simulink model "model_LMPC_yawVarFakeRelative"  (R2024b)
settings: Solver=VariableStepAuto  StartTime=0.0  StopTime=100  RelTol=1e-3
undefined symbols (not defined in the file): boat, boat_wave_Torque, boatModels, drone, environment, settings
libraries: mpclib x4, sharedtransform x3, utils x1, uavutilslib x1
settings Model: Creator=domac  LastModifiedBy=domac

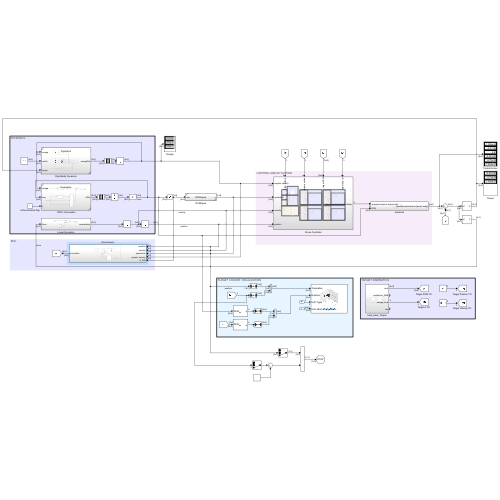
[thumbnail: Simulink's stored preview of the top-level diagram]
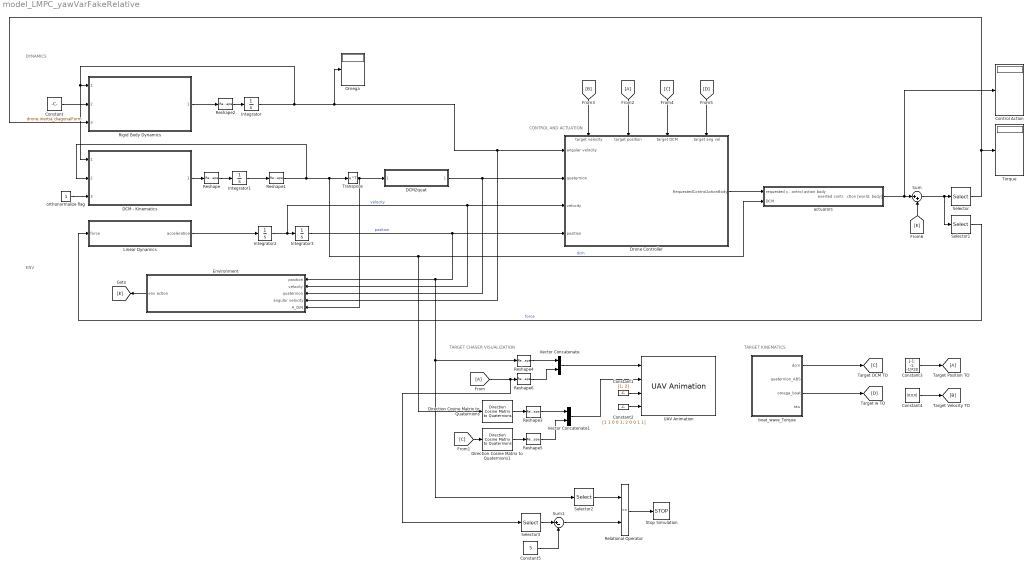
== system model_LMPC_yawVarFakeRelative ==
  note: TARGET CHASER VISUALIZATION
  note: CONTROL AND ACTUATION
  note: DYNAMICS
  note: TARGET KINEMATICS
  note: ENV
  " DCM - Kinematics" : Subsystem  ReferencedSubsystem=Kinematics
  Constant : Constant  Value=drone.inertia_diagonalForm  VectorParams1D=off
  Constant1 : Constant  Value=[1; 2]
  Constant2 : Constant  Value=[1 1 0 0 1; 2 0 0 1 1]
  Constant3 : Constant  Value=[-1; -1; -1]*20
  Constant4 : Constant  Value=[0;0;0]
  Constant5 : Constant  Value=5
  Control Action : Display
  DCM2quat : Subsystem  ReferencedSubsystem=DCM2quat
  Direction Cosine Matrix to Quaternions : sharedtransform/Direction Cosine Matrix  to Quaternions  aMode=0  action=None  tolerance=eps(2)
      settings: LibrarySourceBlock=|
      | aerolibtransform2/Direction Cosine Matrix
      | to Quaternions
  Direction Cosine Matrix to Quaternions1 : sharedtransform/Direction Cosine Matrix  to Quaternions  aMode=0  action=None  tolerance=eps(2)
      settings: LibrarySourceBlock=|
      | aerolibtransform2/Direction Cosine Matrix
      | to Quaternions
  Drone Controller : Subsystem
      settings: PortSchema="{\"entries\":[{\"content\":{\"sides\":[{\"content\":{\"connectorIds\":[\"In1\",\"In2\",\"In3\",\"In4\"]},\"type\":\"ConnectorPlacement.EquallySpacedRectSide\",\"uuid\":\"5cbf5d97-798f-4abe-9063-7d9475aab2f7\"},{\"content\":{\"connectorIds\":[\"Out1\"],\"side\":\"RIGHT\"},\"type\":\"ConnectorPlacement.EquallySpacedRectSide\",\"uuid\":\"8e1c1ff5-210e-451e-9bb4-b2ea9c687a0c\"},{\"content\":{\"connectorIds\":[\"In5\",\"In6\",\"In7\",\"In8\"],\"side\":\"TOP\"},\"type\":\"ConnectorPlacement.EquallySpacedRectSide\",\"uuid\":\"7263c23d-5bc0-464e-848c-51e45572c4cc\"}]},\"type\":\"ConnectorPlacement.EquallySpacedConnector\",\"uuid\":\"7a6c5e6f-7804-4a94-a46d-c2acf2bd8613\"}],\"packageUris\":[\"http://schema.mathworks.com/mf0/Connector/R2020b\"],\"version\":\"1.0\"}"
  Environment : Subsystem
  From : From
  From2 : From
  Integrator : Integrator  InitialCondition=drone.w0
  Integrator1 : Integrator  InitialCondition=[drone.initialDCM(:,1); drone.initialDCM(:,2); drone.initialDCM(:,3)]
  Integrator2 : Integrator  InitialCondition=drone.v0
  Integrator3 : Integrator  InitialCondition=drone.x0
  Linear Dynamics : Subsystem
  Omega : Display
  Relational Operator : RelationalOperator  Operator=<=  OutDataTypeStr=boolean  RndMeth=Simplest  InputSameDT=off
  Reshape : Reshape  OutputDimensionality=Column vector (2-D)
  Reshape1 : Reshape  OutputDimensionality=Customize  OutputDimensions=[3, 3]
  Reshape2 : Reshape  OutputDimensionality=Column vector (2-D)
  Reshape{3..6} (4 alike) : Reshape  OutputDimensionality=Row vector (2-D)
  Rigid Body Dynamics : Subsystem  ReferencedSubsystem=Dynamics
  Selector : Selector  InputPortWidth=6  IndexOptions=Index vector (dialog)  Indices=[4 5 6]  OutputSizes=1
  Selector1 : Selector  InputPortWidth=6  IndexOptions=Index vector (dialog)  Indices=[1 2 3]  OutputSizes=1
  Selector2 : Selector  InputPortWidth=3  IndexOptions=Index vector (dialog)  Indices=3  OutputSizes=1
  Selector3 : Selector  InputPortWidth=3  IndexOptions=Index vector (dialog)  Indices=3  OutputSizes=1
  Stop Simulation : Stop
  Sum : Sum  Inputs=|++
  Sum1 : Sum  Inputs=|+-
  Target Position TO : Goto
  Torque : Display
  Transpose : Math  Operator=transpose
  UAV Animation : uavutilslib/UAV Animation  NumUAV=2  DynamicUAVConfig=on  UAVType=Multirotor  UAVSize=1  UAVColor=[1 0 0]  UAVTrajectoryAlpha=1  InertialZDirection=Up  RotationFormat=Quaternion  DrawMarkers=off  SampleTime=0.2
  Vector Concatenate : Concatenate  Mode=Multidimensional array
  Vector Concatenate1 : Concatenate  Mode=Multidimensional array
  actuarors : Subsystem
  boat_wave_Torque : Subsystem  AncestorBlock=boatModels/boat_wave_Torque
  orthonormalize flag : Constant
  wires:
  Constant/1 -> Rigid Body Dynamics/2
  Integrator1/1 -> Reshape1/1
  DCM2quat/1 -> Drone Controller/2(quaternion), Environment/3(quaternion)
  [D] -> Drone Controller/8(target ang vel)
  Vector Concatenate/1 -> UAV Animation/1
  Reshape4/1 -> Vector Concatenate/1
  From2/1 -> Drone Controller/6(target position)
  Vector Concatenate1/1 -> UAV Animation/2
  orthonormalize flag/1 -> " DCM - Kinematics"/3
  Direction Cosine Matrix to Quaternions/1 -> Reshape3/1
  Sum/1 -> Selector/1, Selector1/1
  Reshape5/1 -> Vector Concatenate1/2
  Reshape6/1 -> Vector Concatenate/2
  actuarors/1(exerted control action [world; body]) -> Control Action/1, Sum/1
  [B] -> Drone Controller/5(target velocity)
  Selector1/1 -> Linear Dynamics/1(force)  "force"
  Reshape/1 -> Integrator1/1
  Reshape1/1 -> " DCM - Kinematics"/2, Direction Cosine Matrix to Quaternions/1, actuarors/2(DCM), Transpose/1  "dcm"
  Constant1/1 -> UAV Animation/3
  [C] -> Drone Controller/7(target DCM)
  [C] -> Direction Cosine Matrix to Quaternions1/1
  Selector/1 -> Rigid Body Dynamics/3, Torque/1
  From/1 -> Selector3/1, Reshape6/1
  Reshape2/1 -> Integrator/1
  Transpose/1 -> Environment/5(A_D/N), DCM2quat/1
  Rigid Body Dynamics/1 -> Reshape2/1
  Integrator3/1 -> Environment/1(position), Reshape4/1, Selector2/1, Drone Controller/4("position ")  "position"
  Integrator2/1 -> Drone Controller/3(velocity), Environment/2(velocity), Integrator3/1  "velocity"
  [E] -> Sum/2
  " DCM - Kinematics"/1 -> Reshape/1
  Environment/1(env action) -> [E]
  Direction Cosine Matrix to Quaternions1/1 -> Reshape5/1
  Integrator/1 -> " DCM - Kinematics"/1, Rigid Body Dynamics/1, Omega/1, Drone Controller/1(angular velocity), Environment/4(angular velocity)
  Reshape3/1 -> Vector Concatenate1/1
  Linear Dynamics/1(acceleration) -> Integrator2/1
  Constant2/1 -> UAV Animation/4
  boat_wave_Torque/1(dcm) -> [C]
  boat_wave_Torque/3(omega_boat) -> [D]
  Constant4/1 -> [B]
  Constant3/1 -> Target Position TO/1
  Drone Controller/1(RequestedControlActionBody) -> actuarors/1(requested control action body)
  Selector2/1 -> Relational Operator/1
  Selector3/1 -> Sum1/1
  Constant5/1 -> Sum1/2
  Sum1/1 -> Relational Operator/2
  Relational Operator/1 -> Stop Simulation/1

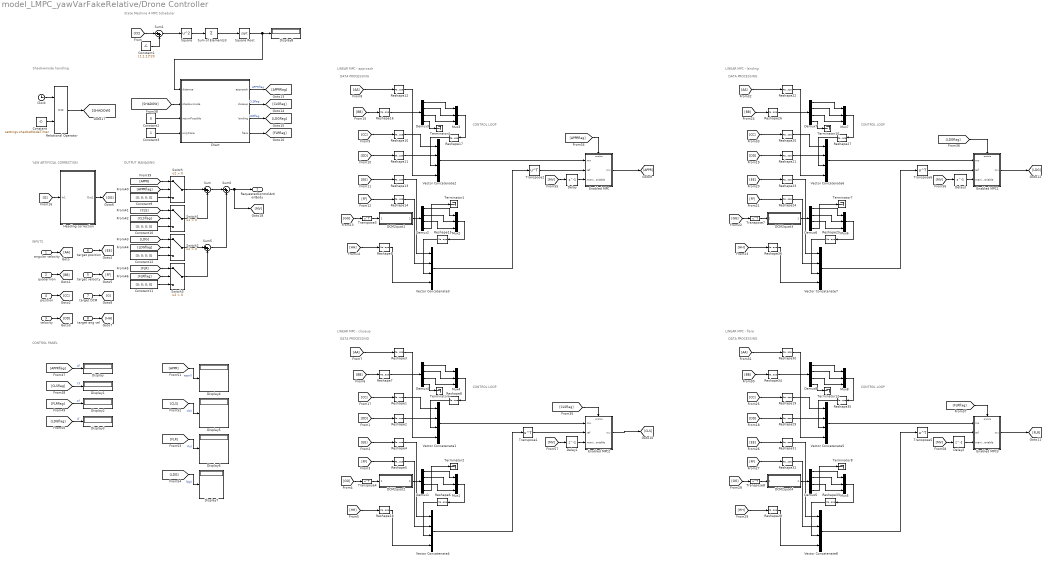
== system model_LMPC_yawVarFakeRelative/Drone Controller ==
  note: CONTROL PANEL
  note: OUTPUT MANAGING
  note: Shadowmode handling
  note: State Machine 4 MPC Scheduler
  note: YAW ARTIFICIAL CORRECTION
  note: INPUTS
  note: DATA PROCESSING
  note: CONTROL LOOP
  note: LINEAR MPC - approach
  note: DATA PROCESSING
  note: CONTROL LOOP
  note: LINEAR MPC - closeup
  note: LINEAR MPC - flare
  note: DATA PROCESSING
  note: CONTROL LOOP
  note: DATA PROCESSING
  note: CONTROL LOOP
  note: LINEAR MPC - landing
  angular velocity : Inport
  quaternion : Inport  Port=2
  velocity : Inport  Port=3
  "position " : Inport  Port=4
  target velocity : Inport  Port=5
  target position : Inport  Port=6
  target DCM : Inport  Port=7
  target ang vel : Inport  Port=8
  Chart : Stateflow chart  TreatAsAtomicUnit=on
  Clock : Clock
  Constant : Constant  Value=settings.shadowModeTimer
  Constant1 : Constant  Value=[1;1;1]*20
  Constant{9..12} (4 alike) : Constant  Value=[0; 0; 0; 0]
  Constant2 : Constant  Value=0
  Constant3 : Constant
  DCM2quat{1..4} (4 alike) : Subsystem  ReferencedSubsystem=DCM2quat
  Delay{,1..3} (4 alike) : Delay  DelayLength=1
  Demux{1..8} (8 alike) : Demux
  Display{,1..8} (9 alike) : Display
  Enabled MPC : Subsystem  TreatAsAtomicUnit=on
  Enabled MPC1 : Subsystem  TreatAsAtomicUnit=on
  Enabled MPC2 : Subsystem  TreatAsAtomicUnit=on
  Enabled MPC3 : Subsystem  TreatAsAtomicUnit=on
  Heading correction : Subsystem
  Mux{1..8} (8 alike) : Mux  Inputs=3
  Relational Operator : RelationalOperator  Operator=<=  OutDataTypeStr=boolean  RndMeth=Simplest  InputSameDT=off
  Reshape{1..36} (36 alike) : Reshape  OutputDimensionality=Column vector (2-D)
  Square : Math  Operator=square
  Square Root : Sqrt
  Sum{,1,5..6} (4 alike) : Sum  Inputs=|++
  Sum of Elements3 : Sum  Inputs=+
  Switch{,1..3} (4 alike) : Switch  Criteria=u2 > Threshold  SaturateOnIntegerOverflow=off  InputSameDT=off
  Terminator{1..2,4,6..8,10,12} (8 alike) : Terminator
  Transpose{1..8} (8 alike) : Math  Operator=transpose
  Vector Concatenate{1..8} (8 alike) : Concatenate  NumInputs=4
  RequestedControlActionBody : Outport
  wires:
  Transpose2/1 -> Enabled MPC/2(ref)
  Vector Concatenate2/1 -> Enabled MPC/1(mo)
  [FF] -> Reshape14/1
  Demux2/2 -> Mux2/2
  Reshape10/1 -> Vector Concatenate2/1
  Reshape12/1 -> Vector Concatenate2/4
  Reshape15/1 -> Vector Concatenate3/3
  [HH] -> Reshape9/1
  Vector Concatenate3/1 -> Transpose2/1
  Reshape9/1 -> Vector Concatenate3/4
  Demux2/1 -> Mux2/1
  [CC] -> Reshape10/1
  DCM2quat1/1 -> Demux2/1
  [BB] -> Reshape16/1
  Reshape11/1 -> Vector Concatenate2/2
  Reshape17/1 -> Vector Concatenate2/3
  [DD] -> Reshape11/1
  Reshape14/1 -> Vector Concatenate3/2
  Mux3/1 -> Reshape17/1
  [EE] -> Reshape13/1
  Mux2/1 -> Reshape15/1
  Reshape16/1 -> Demux3/1
  Demux3/1 -> Mux3/1
  [AA] -> Reshape12/1
  Demux3/4 -> Terminator4/1
  Demux3/3 -> Mux3/3
  Demux2/4 -> Terminator1/1
  Transpose3/1 -> DCM2quat1/1
  Demux3/2 -> Mux3/2
  Reshape13/1 -> Vector Concatenate3/1
  Demux2/3 -> Mux2/3
  angular velocity/1 -> [AA]
  quaternion/1 -> [BB]
  velocity/1 -> [DD]
  "position "/1 -> [CC]
  target position/1 -> [EE]
  target velocity/1 -> [FF]
  target ang vel/1 -> [HH]
  [GG] -> Transpose3/1
  target DCM/1 -> [G]
  [G] -> Heading correction/1(In1)
  Heading correction/1(Out1) -> [GG]
  Enabled MPC/1(mv) -> [APPR]
  Vector Concatenate1/1 -> Enabled MPC2/1(mo)
  DCM2quat2/1 -> Demux1/1
  [BB] -> Reshape7/1
  Transpose1/1 -> Enabled MPC2/2(ref)
  Reshape8/1 -> Vector Concatenate1/3
  Enabled MPC2/1(mv) -> [CLS]
  [GG] -> Transpose4/1
  [CC] -> Reshape1/1
  Demux4/4 -> Terminator6/1
  [HH] -> Reshape18/1
  Demux1/4 -> Terminator2/1
  Reshape6/1 -> Vector Concatenate4/3
  Demux4/3 -> Mux4/3
  Demux4/2 -> Mux4/2
  Mux4/1 -> Reshape8/1
  [EE] -> Reshape4/1
  Reshape7/1 -> Demux4/1
  Demux1/2 -> Mux1/2
  Transpose4/1 -> DCM2quat2/1
  Mux1/1 -> Reshape6/1
  [FF] -> Reshape5/1
  Reshape5/1 -> Vector Concatenate4/2
  Reshape3/1 -> Vector Concatenate1/4
  Reshape1/1 -> Vector Concatenate1/1
  Reshape2/1 -> Vector Concatenate1/2
  Demux1/3 -> Mux1/3
  [DD] -> Reshape2/1
  Reshape4/1 -> Vector Concatenate4/1
  Vector Concatenate4/1 -> Transpose1/1
  Demux4/1 -> Mux4/1
  Reshape18/1 -> Vector Concatenate4/4
  [AA] -> Reshape3/1
  Demux1/1 -> Mux1/1
  Vector Concatenate6/1 -> Enabled MPC1/1(mo)
  Enabled MPC1/1(mv) -> [LDG]
  Demux5/1 -> Mux5/1
  [AA] -> Reshape30/1
  Transpose6/1 -> Enabled MPC1/2(ref)
  Demux5/3 -> Mux5/3
  [DD] -> Reshape29/1
  Demux8/1 -> Mux8/1
  Reshape31/1 -> Vector Concatenate8/1
  Vector Concatenate8/1 -> Transpose5/1
  Reshape30/1 -> Vector Concatenate5/4
  Mux5/1 -> Reshape33/1
  Demux8/3 -> Mux8/3
  Demux5/2 -> Mux5/2
  Reshape28/1 -> Vector Concatenate8/4
  Mux8/1 -> Reshape35/1
  [FF] -> Reshape32/1
  [CC] -> Reshape19/1
  Reshape19/1 -> Vector Concatenate5/1
  [BB] -> Reshape34/1
  DCM2quat4/1 -> Demux5/1
  DCM2quat3/1 -> Demux6/1
  Reshape33/1 -> Vector Concatenate8/3
  Reshape35/1 -> Vector Concatenate5/3
  [BB] -> Reshape26/1
  Reshape27/1 -> Vector Concatenate6/3
  [GG] -> Transpose7/1
  Demux8/2 -> Mux8/2
  [CC] -> Reshape20/1
  Demux7/4 -> Terminator10/1
  Transpose8/1 -> DCM2quat4/1
  [HH] -> Reshape28/1
  [HH] -> Reshape36/1
  Demux8/4 -> Terminator12/1
  Reshape29/1 -> Vector Concatenate5/2
  Demux6/4 -> Terminator7/1
  Reshape25/1 -> Vector Concatenate7/3
  Demux7/3 -> Mux7/3
  [EE] -> Reshape31/1
  Demux7/2 -> Mux7/2
  Mux7/1 -> Reshape27/1
  [EE] -> Reshape23/1
  Vector Concatenate5/1 -> Enabled MPC3/1(mo)
  Reshape26/1 -> Demux7/1
  Reshape34/1 -> Demux8/1
  Transpose5/1 -> Enabled MPC3/2(ref)
  Demux6/2 -> Mux6/2
  Transpose7/1 -> DCM2quat3/1
  Mux6/1 -> Reshape25/1
  [FF] -> Reshape24/1
  Reshape24/1 -> Vector Concatenate7/2
  Reshape22/1 -> Vector Concatenate6/4
  Reshape20/1 -> Vector Concatenate6/1
  Reshape21/1 -> Vector Concatenate6/2
  Enabled MPC3/1(mv) -> [FLR]
  Demux6/3 -> Mux6/3
  [DD] -> Reshape21/1
  Reshape23/1 -> Vector Concatenate7/1
  Vector Concatenate7/1 -> Transpose6/1
  [GG] -> Transpose8/1
  Demux7/1 -> Mux7/1
  Demux5/4 -> Terminator8/1
  Reshape36/1 -> Vector Concatenate7/4
  [AA] -> Reshape22/1
  Reshape32/1 -> Vector Concatenate8/2
  Demux6/1 -> Mux6/1
  Chart/1(approach) -> [APPRflag]  "APPRflag"
  Chart/2(closeup) -> [CLSflag]  "CLSflag"
  Chart/3(landing) -> [LDGflag]  "LDGflag"
  Chart/4(flare) -> [FLRflag]
  [APPRflag] -> Enabled MPC/Enable
  [CLSflag] -> Enabled MPC2/Enable
  [LDGflag] -> Enabled MPC1/Enable
  [FLRflag] -> Enabled MPC3/Enable
  [SHADOW] -> Chart/2(shadowmode)
  Clock/1 -> Relational Operator/1
  Constant/1 -> Relational Operator/2
  Relational Operator/1 -> [SHADOW]
  [APPR] -> Switch/1
  [APPRflag] -> Switch/2
  Constant9/1 -> Switch/3
  [CLS] -> Switch1/1
  [CLSflag] -> Switch1/2
  Constant10/1 -> Switch1/3
  [LDG] -> Switch2/1
  Constant11/1 -> Switch3/3
  [FLR] -> Switch3/1
  [LDGflag] -> Switch2/2
  [FLRflag] -> Switch3/2
  Constant12/1 -> Switch2/3
  Switch/1 -> Sum/1
  Switch1/1 -> Sum/2
  Switch3/1 -> Sum5/2
  Switch2/1 -> Sum5/1
  Sum/1 -> Sum6/1
  Sum5/1 -> Sum6/2
  Sum6/1 -> [MV], RequestedControlActionBody/1
  Square/1 -> Sum of Elements3/1
  Sum of Elements3/1 -> Square Root/1
  Square Root/1 -> Display8/1, Chart/1(distance)
  [APPRflag] -> Display/1  "Af"
  [CLSflag] -> Display1/1  "Cf"
  [FLRflag] -> Display2/1  "Ff"
  [LDGflag] -> Display3/1  "Lf"
  [LDG] -> Display7/1  "ldgU"
  [FLR] -> Display6/1  "flrU"
  [APPR] -> Display4/1  "apprU"
  [CLS] -> Display5/1  "clsU"
  [CC] -> Sum1/1
  Sum1/1 -> Square/1
  Constant1/1 -> Sum1/2
  [MV] -> Delay/1
  [MV] -> Delay3/1
  [MV] -> Delay1/1
  [MV] -> Delay2/1
  Delay/1 -> Enabled MPC/3(manipulated variable)
  Delay1/1 -> Enabled MPC2/3(manipulated variable)
  Delay2/1 -> Enabled MPC3/3(manipulated variable)
  Delay3/1 -> Enabled MPC1/3(manipulated variable)
  Constant2/1 -> Chart/3(returnPossible)
  Constant3/1 -> Chart/4(onlyFlare)

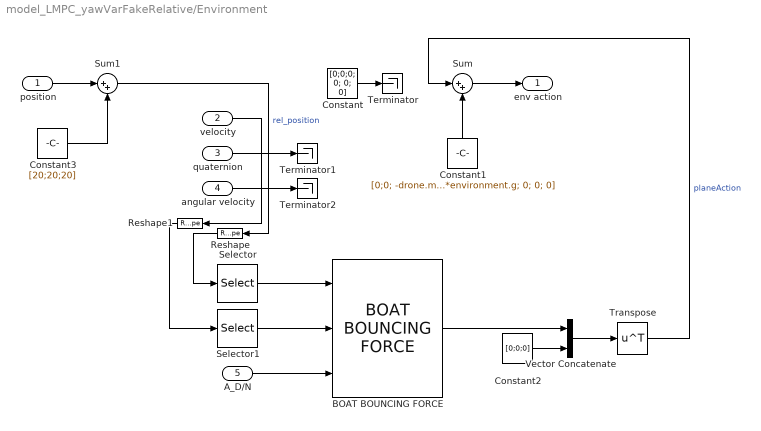
== system model_LMPC_yawVarFakeRelative/Environment ==
  position : Inport
  velocity : Inport  Port=2
  quaternion : Inport  Port=3
  angular velocity : Inport  Port=4
  A_D/N : Inport  Port=5
  BOAT BOUNCING FORCE : utils/BOAT BOUNCING FORCE  SystemSampleTime=-1  VariantActivationTime=update diagram  AllowFlexibleInterface=on  Latency=0  AutoFrameSizeCalculation=off
  Constant : Constant  Value=[0;0;0; 0; 0; 0]
  Constant1 : Constant  Value=[0;0; -drone.m*environment.g; 0; 0; 0]
  Constant2 : Constant  Value=[0;0;0]
  Constant3 : Constant  Value=[20;20;20]
  Reshape : Reshape  OutputDimensionality=Column vector (2-D)
  Reshape1 : Reshape  OutputDimensionality=Column vector (2-D)
  Selector : Selector  NumberOfDimensions=2  InputPortWidth=3  IndexOptions=Index vector (dialog),Index vector (dialog)  Indices=[3],1  OutputSizes=1,1
  Selector1 : Selector  NumberOfDimensions=2  InputPortWidth=3  IndexOptions=Index vector (dialog),Index vector (dialog)  Indices=[3],1  OutputSizes=1,1
  Sum : Sum  Inputs=|++
  Sum1 : Sum  Inputs=|++
  Terminator : Terminator
  Terminator1 : Terminator
  Terminator2 : Terminator
  Transpose : Math  Operator=transpose
  Vector Concatenate : Concatenate
  env action : Outport
  wires:
  velocity/1 -> Reshape1/1
  angular velocity/1 -> Terminator2/1
  quaternion/1 -> Terminator1/1
  Constant1/1 -> Sum/2
  Sum/1 -> env action/1
  A_D/N/1 -> BOAT BOUNCING FORCE/3
  Selector1/1 -> BOAT BOUNCING FORCE/2
  Selector/1 -> BOAT BOUNCING FORCE/1
  BOAT BOUNCING FORCE/1 -> Vector Concatenate/1
  Constant/1 -> Terminator/1
  Constant2/1 -> Vector Concatenate/2
  Vector Concatenate/1 -> Transpose/1
  Reshape/1 -> Selector/1
  Reshape1/1 -> Selector1/1
  Transpose/1 -> Sum/1  "planeAction"
  Constant3/1 -> Sum1/2
  Sum1/1 -> Reshape/1  "rel_position"
  position/1 -> Sum1/1

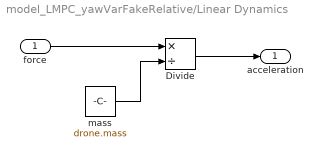
== system model_LMPC_yawVarFakeRelative/Linear Dynamics ==
  force : Inport
  Divide : Product  Inputs=*/
  mass : Constant  Value=drone.mass
  acceleration : Outport
  wires:
  force/1 -> Divide/1
  mass/1 -> Divide/2
  Divide/1 -> acceleration/1

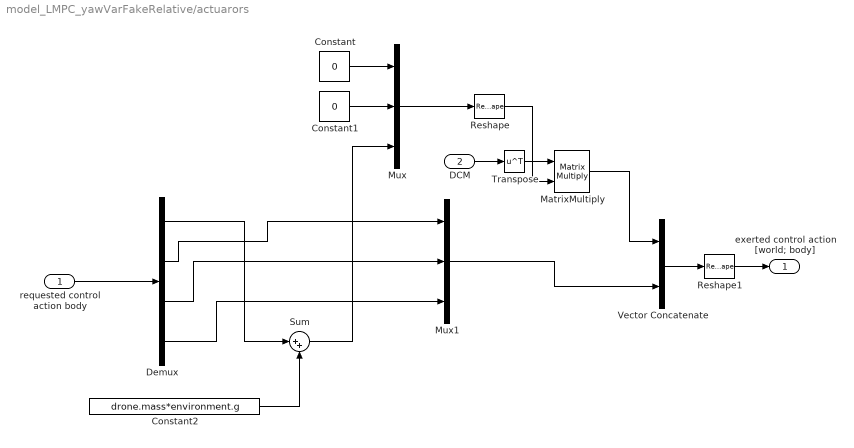
== system model_LMPC_yawVarFakeRelative/actuarors ==
  requested control action body : Inport
  DCM : Inport  Port=2
  Constant : Constant  Value=0
  Constant1 : Constant  Value=0
  Constant2 : Constant  Value=drone.mass*environment.g
  Demux : Demux
  MatrixMultiply : Product  Multiplication=Matrix(*)
  Mux : Mux  Inputs=3
  Mux1 : Mux  Inputs=3
  Reshape : Reshape  OutputDimensionality=Column vector (2-D)
  Reshape1 : Reshape  OutputDimensionality=Column vector (2-D)
  Sum : Sum  Inputs=|++
  Transpose : Math  Operator=transpose
  Vector Concatenate : Concatenate
  exerted control action [world; body] : Outport
  wires:
  Constant/1 -> Mux/1
  Constant1/1 -> Mux/2
  requested control action body/1 -> Demux/1
  DCM/1 -> Transpose/1
  Mux/1 -> Reshape/1
  Reshape/1 -> MatrixMultiply/2
  MatrixMultiply/1 -> Vector Concatenate/1
  Mux1/1 -> Vector Concatenate/2
  Vector Concatenate/1 -> Reshape1/1
  Reshape1/1 -> exerted control action [world; body]/1
  Sum/1 -> Mux/3
  Constant2/1 -> Sum/2
  Demux/1 -> Sum/1
  Demux/4 -> Mux1/3
  Demux/3 -> Mux1/2
  Demux/2 -> Mux1/1
  Transpose/1 -> MatrixMultiply/1

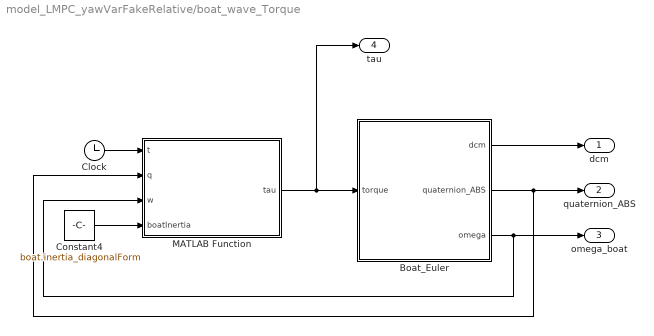
== system model_LMPC_yawVarFakeRelative/boat_wave_Torque ==
  Boat_Euler : Subsystem
  Clock : Clock
  Constant4 : Constant  Value=boat.inertia_diagonalForm
  MATLAB Function : MATLAB Function  TreatAsAtomicUnit=on
  dcm : Outport
  quaternion_ABS : Outport  Port=2
  omega_boat : Outport  Port=3
  tau : Outport  Port=4
  wires:
  Boat_Euler/1(dcm) -> dcm/1
  Clock/1 -> MATLAB Function/1(t)
  Boat_Euler/2(quaternion_ABS) -> MATLAB Function/2(q), quaternion_ABS/1
  Constant4/1 -> MATLAB Function/4(boatInertia)
  Boat_Euler/3(omega) -> MATLAB Function/3(w), omega_boat/1
  MATLAB Function/1(tau) -> Boat_Euler/1(torque), tau/1

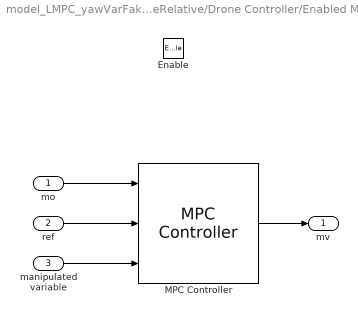
== system model_LMPC_yawVarFakeRelative/Drone Controller/Enabled MPC ==
  mo : Inport
  ref : Inport  Port=2
  manipulated variable : Inport  Port=3
  Enable : EnablePort
  MPC Controller : mpclib/MPC Controller  SCDEnableBlockLinearizationSpecification=on  mpcobj=mpcAPPROACH  is_multiple=0  enable_value=0  return_u0=off  updateMPCinCallerWorkspace=on  md_inport=off  mv_inport=on  uref_inport=off  return_cost=off  return_mvseq=off  return_qpstatus=off  return_xseq=off  return_state=off  return_ovseq=off  state_inport=on  umin_inport=off  umax_inport=off  ymin_inport=off  ymax_inport=off  cc_inport=off  ywt_inport=off  uwt_inport=off  duwt_inport=off  rhoeps_inport=off  pm_inport=off  MaximumP=10  HorizonChoice=FixedHorizon  n_ts=0.025  n_p=100  n_mv=4  n_md=0  n_ud=0  n_mo=12  n_uo=0  BlockDataType=double  SampleTimeInherited=off  switch_inport=off
  mv : Outport  OutputWhenDisabled=reset  InitialOutput=[0;0;0;0]
  wires:
  MPC Controller/1 -> mv/1
  ref/1 -> MPC Controller/2
  mo/1 -> MPC Controller/1
  manipulated variable/1 -> MPC Controller/3

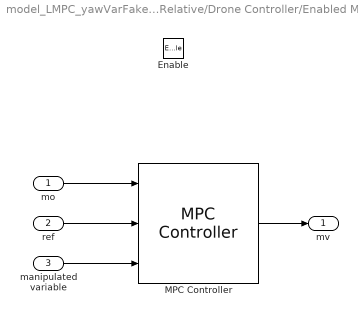
== system model_LMPC_yawVarFakeRelative/Drone Controller/Enabled MPC1 ==
  mo : Inport
  ref : Inport  Port=2
  manipulated variable : Inport  Port=3
  Enable : EnablePort
  MPC Controller : mpclib/MPC Controller  SCDEnableBlockLinearizationSpecification=on  mpcobj=mpcLANDING  is_multiple=0  enable_value=0  return_u0=off  updateMPCinCallerWorkspace=on  md_inport=off  mv_inport=on  uref_inport=off  return_cost=off  return_mvseq=off  return_qpstatus=off  return_xseq=off  return_state=off  return_ovseq=off  state_inport=on  umin_inport=off  umax_inport=off  ymin_inport=off  ymax_inport=off  cc_inport=off  ywt_inport=off  uwt_inport=off  duwt_inport=off  rhoeps_inport=off  pm_inport=off  MaximumP=10  HorizonChoice=FixedHorizon  n_ts=0.025  n_p=100  n_mv=4  n_md=0  n_ud=0  n_mo=12  n_uo=0  BlockDataType=double  SampleTimeInherited=off  switch_inport=off
  mv : Outport  OutputWhenDisabled=reset  InitialOutput=[0;0;0;0]
  wires:
  MPC Controller/1 -> mv/1
  ref/1 -> MPC Controller/2
  mo/1 -> MPC Controller/1
  manipulated variable/1 -> MPC Controller/3

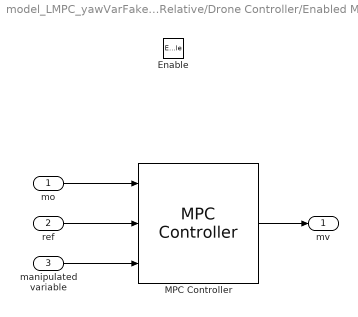
== system model_LMPC_yawVarFakeRelative/Drone Controller/Enabled MPC2 ==
  mo : Inport
  ref : Inport  Port=2
  manipulated variable : Inport  Port=3
  Enable : EnablePort
  MPC Controller : mpclib/MPC Controller  SCDEnableBlockLinearizationSpecification=on  mpcobj=mpcCLOSEUP  is_multiple=0  enable_value=0  return_u0=off  updateMPCinCallerWorkspace=on  md_inport=off  mv_inport=on  uref_inport=off  return_cost=off  return_mvseq=off  return_qpstatus=off  return_xseq=off  return_state=off  return_ovseq=off  state_inport=on  umin_inport=off  umax_inport=off  ymin_inport=off  ymax_inport=off  cc_inport=off  ywt_inport=off  uwt_inport=off  duwt_inport=off  rhoeps_inport=off  pm_inport=off  MaximumP=10  HorizonChoice=FixedHorizon  n_ts=0.025  n_p=100  n_mv=4  n_md=0  n_ud=0  n_mo=12  n_uo=0  BlockDataType=double  SampleTimeInherited=off  switch_inport=off
  mv : Outport  OutputWhenDisabled=reset  InitialOutput=[0;0;0;0]
  wires:
  MPC Controller/1 -> mv/1
  ref/1 -> MPC Controller/2
  mo/1 -> MPC Controller/1
  manipulated variable/1 -> MPC Controller/3

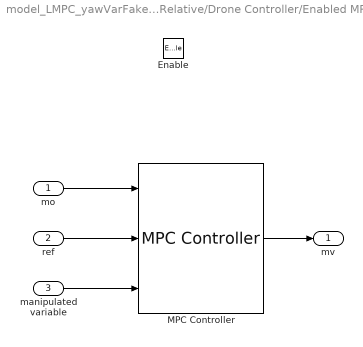
== system model_LMPC_yawVarFakeRelative/Drone Controller/Enabled MPC3 ==
  mo : Inport
  ref : Inport  Port=2
  manipulated variable : Inport  Port=3
  Enable : EnablePort
  MPC Controller : mpclib/MPC Controller  SCDEnableBlockLinearizationSpecification=on  mpcobj=mpcFLARE  is_multiple=0  enable_value=0  return_u0=off  updateMPCinCallerWorkspace=on  md_inport=off  mv_inport=on  uref_inport=off  return_cost=off  return_mvseq=off  return_qpstatus=off  return_xseq=off  return_state=off  return_ovseq=off  state_inport=on  umin_inport=off  umax_inport=off  ymin_inport=off  ymax_inport=off  cc_inport=off  ywt_inport=off  uwt_inport=off  duwt_inport=off  rhoeps_inport=off  pm_inport=off  MaximumP=10  HorizonChoice=FixedHorizon  n_ts=0.025  n_p=100  n_mv=4  n_md=0  n_ud=0  n_mo=12  n_uo=0  BlockDataType=double  SampleTimeInherited=off  switch_inport=off
  mv : Outport  OutputWhenDisabled=reset  InitialOutput=[0;0;0;0]
  wires:
  MPC Controller/1 -> mv/1
  ref/1 -> MPC Controller/2
  manipulated variable/1 -> MPC Controller/3
  mo/1 -> MPC Controller/1

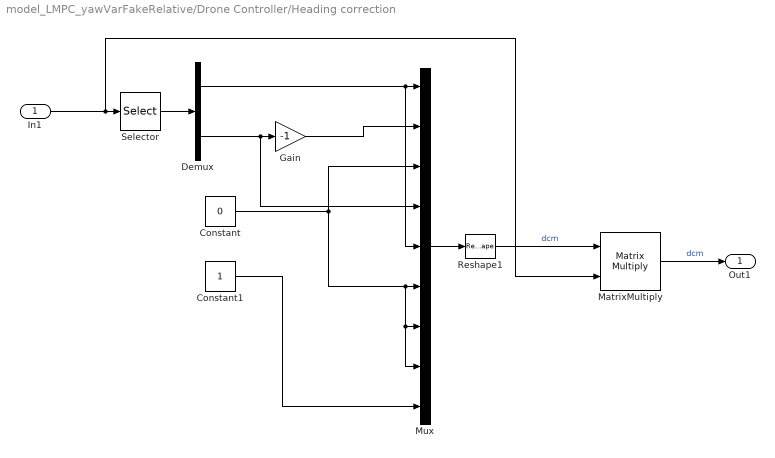
== system model_LMPC_yawVarFakeRelative/Drone Controller/Heading correction ==
  In1 : Inport
  Constant : Constant  Value=0
  Constant1 : Constant
  Demux : Demux  Outputs=2
  Gain : Gain  Gain=-1
  MatrixMultiply : Product  Multiplication=Matrix(*)
  Mux : Mux  Inputs=9
  Reshape1 : Reshape  OutputDimensionality=Customize  OutputDimensions=[3, 3]
  Selector : Selector  NumberOfDimensions=2  InputPortWidth=3  IndexOptions=Index vector (dialog),Index vector (dialog)  Indices=1,[1 2]  OutputSizes=1,1
  Out1 : Outport
  wires:
  MatrixMultiply/1 -> Out1/1  "dcm"
  In1/1 -> MatrixMultiply/2, Selector/1
  Selector/1 -> Demux/1
  Demux/1 -> Mux/5, Mux/1
  Demux/2 -> Mux/4, Gain/1
  Gain/1 -> Mux/2
  Constant/1 -> Mux/8, Mux/7, Mux/6, Mux/3
  Constant1/1 -> Mux/9
  Mux/1 -> Reshape1/1
  Reshape1/1 -> MatrixMultiply/1  "dcm"

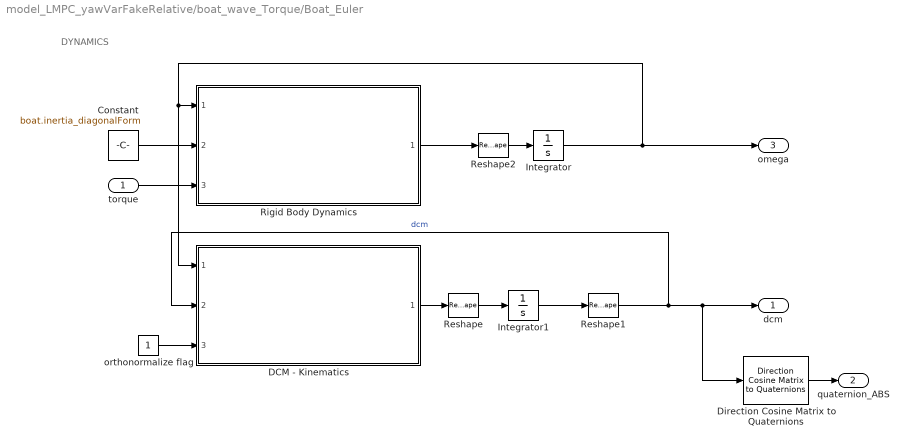
== system model_LMPC_yawVarFakeRelative/boat_wave_Torque/Boat_Euler ==
  note: DYNAMICS
  torque : Inport
  " DCM - Kinematics" : Subsystem  ReferencedSubsystem=Kinematics
  Constant : Constant  Value=boat.inertia_diagonalForm  VectorParams1D=off
  Direction Cosine Matrix to Quaternions : sharedtransform/Direction Cosine Matrix  to Quaternions  aMode=0  action=None  tolerance=eps(2)
  Integrator : Integrator  InitialCondition=boat.w0
  Integrator1 : Integrator  InitialCondition=[boat.initialDCM(:,1); boat.initialDCM(:,2); boat.initialDCM(:,3)]
  Reshape : Reshape  OutputDimensionality=Column vector (2-D)
  Reshape1 : Reshape  OutputDimensionality=Customize  OutputDimensions=[3, 3]
  Reshape2 : Reshape  OutputDimensionality=Column vector (2-D)
  Rigid Body Dynamics : Subsystem  ReferencedSubsystem=Dynamics
  orthonormalize flag : Constant
  dcm : Outport
  quaternion_ABS : Outport  Port=2
  omega : Outport  Port=3
  wires:
  Direction Cosine Matrix to Quaternions/1 -> quaternion_ABS/1
  torque/1 -> Rigid Body Dynamics/3
  Reshape1/1 -> " DCM - Kinematics"/2, dcm/1, Direction Cosine Matrix to Quaternions/1  "dcm"
  Reshape2/1 -> Integrator/1
  Integrator/1 -> Rigid Body Dynamics/1, " DCM - Kinematics"/1, omega/1
  " DCM - Kinematics"/1 -> Reshape/1
  Constant/1 -> Rigid Body Dynamics/2
  Rigid Body Dynamics/1 -> Reshape2/1
  Integrator1/1 -> Reshape1/1
  Reshape/1 -> Integrator1/1
  orthonormalize flag/1 -> " DCM - Kinematics"/3

== matlab function model_LMPC_yawVarFakeRelative/boat_wave_Torque/MATLAB Function ==
  data: t input; tau output; q input; w input; boatInertia input
function tau = waveTorque(t, q, w, boatInertia)
q = q / norm(q);
q0 = q(1); q1 = q(2); q2 = q(3); q3 = q(4);
phi   = atan2(2*(q0*q1 + q2*q3), 1 - 2*(q1^2 + q2^2));
theta = asin(max(-1, min(1, 2*(q0*q2 - q3*q1))));
psi   = atan2(2*(q0*q3 + q1*q2), 1 - 2*(q2^2 + q3^2));

% boat
rho = 1025; g = 9.81;
Vol = 2.0;  GMT = 0.8;  GML = 6.0;
Ixx = boatInertia(1);  Iyy = boatInertia(2);
zr = 0.10;  zp = 0.25;  Bz = 500;

% sea parameters
Hs = 1.0; Tp = 6; gam = 3.3;
chi = 90*pi/180;     
N = 50;

Cphi = rho*g*Vol*GMT;  Cth = rho*g*Vol*GML;
Bphi = 2*zr*sqrt(Cphi*Ixx);  Bth = 2*zp*sqrt(Cth*Iyy);

wp = 2*pi/Tp; wmin = 0.5*wp; wmax = 3*wp; dw = (wmax-wmin)/N;
i = (1:N)';
wi = wmin + (i - 1 + mod(i*0.6180339887,1))*dw;
sig = 0.07 + 0.02*(wi > wp);
S = (5/16)*Hs^2*wp^4./wi.^5 .* exp(-1.25*(wp./wi).^4) ...
    .* gam.^exp(-(wi-wp).^2./(2*sig.^2*wp^2)) * (1-0.287*log(gam));
kai   = (wi.^2/g) .* sqrt(2*S*dw);
phi_i = mod(i*2.399963229728653, 2*pi);

alpha = sum(kai .* sin(wi*t + phi_i));
beta  = chi - psi;

tau = [ -Cphi*(phi   - sin(beta)*alpha) - Bphi*w(1);
        -Cth *(theta - cos(beta)*alpha) - Bth *w(2);
        -Bz*w(3) ];

tau = tau*10;

end

== stateflow chart model_LMPC_yawVarFakeRelative/Drone Controller/Chart ==
  state Shadowmode
  state Approaching
    approach = true;
    closeup = false;
    landing = false;
    flare = false;
  state ClosingUp
    approach = false;
    closeup = true;
    landing = false;
    flare = false;
  state Landing
    approach = false;
    closeup = false;
    landing = true;
    flare = false;
  state Flaring
    approach = false;
    closeup = false;
    landing = false;
    flare = true;
  (default) -> Shadowmode : {flare = false;
      | landing = false;
      | closeup = false;
      | approach = false;}
  Shadowmode -> Flaring [order 2] : [onlyFlare > 0]
  Shadowmode -> Approaching [order 1] : [~shadowmode && onlyFlare]
  Flaring -> Approaching [order 3] : [returnPossible > 0 && distance > scheduler.radius1_out]
  Landing -> Approaching [order 1] : [distance > scheduler.radius2_out && distance > scheduler.radius1_out]
  ClosingUp -> Approaching [order 2] : [distance > scheduler.radius1_out]
  Approaching -> ClosingUp : [distance < scheduler.radius1_in]
  Flaring -> ClosingUp [order 2] : [returnPossible > 0 && distance > scheduler.radius2_out && distance < scheduler.radius1_in]
  Landing -> ClosingUp [order 2] : [distance > scheduler.radius2_out && distance < scheduler.radius1_in]
  ClosingUp -> Landing [order 1] : [distance < scheduler.radius2_in]
  Flaring -> Landing [order 1] : [returnPossible > 0 && distance > scheduler.radius3_out && distance < scheduler.radius2_in]
  Landing -> Flaring [order 3] : [distance < scheduler.radius3_in]
  data: distance input; approach output; closeup output; landing output; flare output; shadowmode input; scheduler parameter; returnPossible input; onlyFlare input
